simulink model "SRA_P2_integrativo"  (R2026b)
settings: Solver=VariableStepAuto  StopTime=100.0
settings Model: Creator=paull  LastModifiedBy=vidal

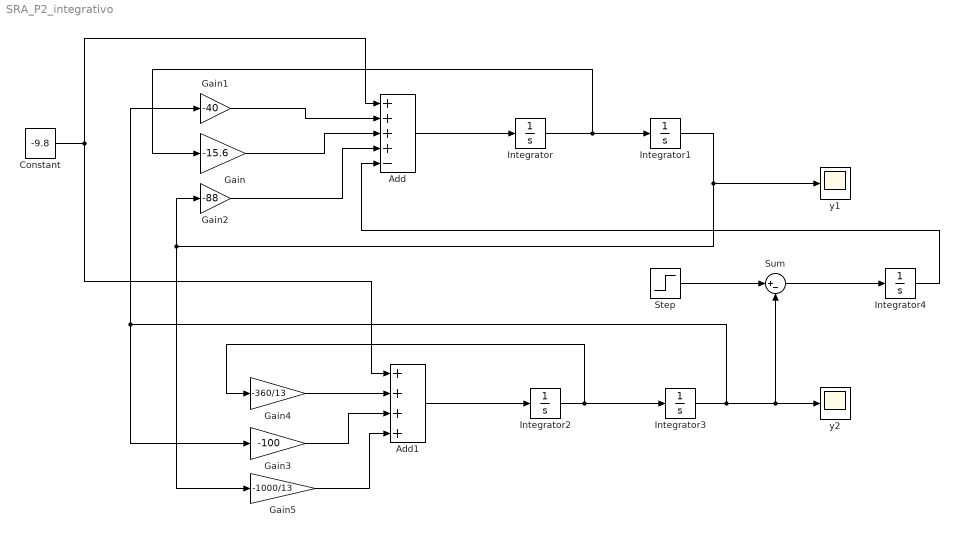
== system SRA_P2_integrativo ==
  Add : Sum  Inputs=++++-
  Add1 : Sum  Inputs=++++
  Constant : Constant  Value=-9.8
  Gain : Gain  Gain=-15.6
  Gain1 : Gain  Gain=-40
  Gain2 : Gain  Gain=-88
  Gain3 : Gain  Gain=-100
  Gain4 : Gain  Gain=-360/13
  Gain5 : Gain  Gain=-1000/13
  Integrator{,1..3} (4 alike) : Integrator
  Integrator4 : Integrator  InitialCondition=5
  Step : Step  Time=0  FinalValue=5  SampleTime=0
  Sum : Sum  Inputs=|+-
  y1 : Scope
      settings: ActiveDisplayYMinimum=4.9714407883892149E+7  ActiveDisplayYMaximum=5.8147941621422969E+7
  y2 : Scope
      settings: ActiveDisplayYMinimum=-10.197831020835464  ActiveDisplayYMaximum=12.323283601082286
  wires:
  Integrator1/1 -> Gain2/1, Gain5/1, y1/1
  Integrator/1 -> Integrator1/1, Gain/1
  Add/1 -> Integrator/1
  Gain2/1 -> Add/4
  Gain/1 -> Add/3
  Integrator3/1 -> Gain3/1, Gain1/1, Sum/2, y2/1
  Integrator2/1 -> Gain4/1, Integrator3/1
  Constant/1 -> Add/1, Add1/1
  Gain1/1 -> Add/2
  Add1/1 -> Integrator2/1
  Gain4/1 -> Add1/2
  Gain3/1 -> Add1/3
  Gain5/1 -> Add1/4
  Sum/1 -> Integrator4/1
  Integrator4/1 -> Add/5
  Step/1 -> Sum/1
